simulink model "EntryExit_ports"  (R2025b)
settings: Solver=FixedStepDiscrete  StartTime=0.0  StopTime=10.0  FixedStep=0.1  RelTol=1e-3  EnableMultiTasking=on
settings Model: Creator=SHG3KOR  LastModifiedBy=CAQ2KOR
settings SolverCC: AlgebraicLoopSolver=TrustRegion  AutoInsertRateTranBlk=on
settings DataIOCC: LimitDataPoints=on
settings OptimizationCC: LifeSpan=inf
settings DebuggingCC: UnconnectedInputMsg=warning  UnconnectedOutputMsg=warning  UnconnectedLineMsg=warning  AllowSymbolicDim=off  SFUnexpectedBacktrackingDiag=warning  SFNoUnconditionalDefaultTransitionDiag=warning  SFExecutionAtInitializationDiag=none  ArithmeticOperatorsInVariantConditions=warning
settings ModelReferenceCC: EnableRefExpFcnMdlSchedulingChecks=on
settings SFSimCC: SimUseLocalCustomCode=off  CustomCodeUndefinedFunction=UseInterfaceOnly
settings RTWCC: RTWUseLocalCustomCode=off  GPUComputeCapability=3.5  DLArmComputeVersion=19.05
settings CodeAppCC: StateflowObjectComments=on
settings GRTTargetCC: TargetLangStandard=C89/C90 (ANSI)
settings ConfigComp: CovMetricSettings=dw  CovSaveCumulativeToWorkspaceVar=on  CovSaveSingleToWorkspaceVar=on  CovExternalEMLEnable=off

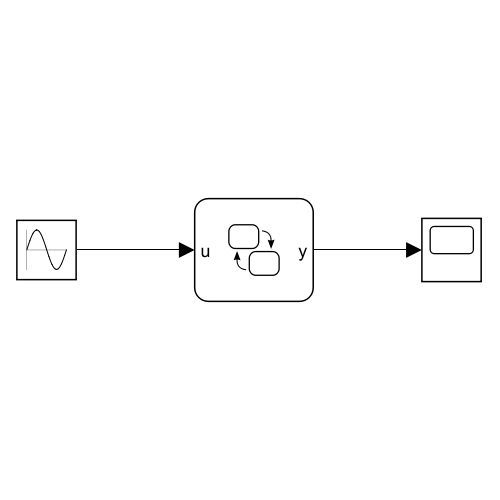
[thumbnail: Simulink's stored preview of the top-level diagram]
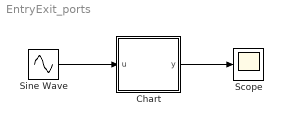
== system EntryExit_ports ==
  Chart : Stateflow chart  TreatAsAtomicUnit=on
  Scope : Scope
      settings: DataLoggingSaveFormat=Array
  Sine Wave : Sin  SampleTime=0
  wires:
  Sine Wave/1 -> Chart/1(u)
  Chart/1(y) -> Scope/1

== stateflow chart EntryExit_ports/Chart ==
  state State1 %State Name
    entry: y = -1; % entry action
    % during:
  (default) -> State1 %State Name
  State1 %State Name -> 9 : [u <= 0]
      | % [transition condition]{action}
  11 -> State1 %State Name
  data: u input; y output
